simulink model "DT_V1_Transformer_Electrical_Healthy"  (R2026a)
settings: Solver=VariableStepAuto  StopTime=0.2
libraries: eeRmsMeasurement x12, nesl_utility x7, ee_lib x6, fl_lib x3

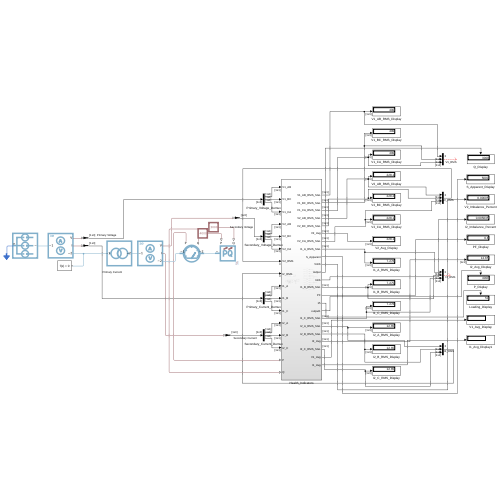
[thumbnail: Simulink's stored preview of the top-level diagram]
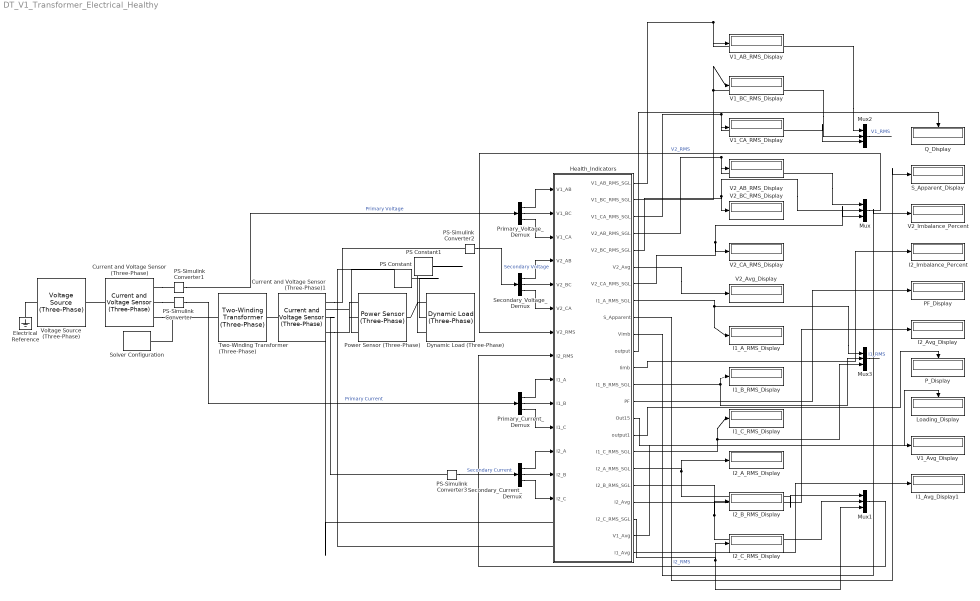
== system DT_V1_Transformer_Electrical_Healthy ==
  Current and Voltage Sensor (Three-Phase) : ee_lib/Sensors & Transducers/Current and Voltage Sensor (Three-Phase)  port_option=ee.enum.threePhasePort.composite  vMeasurementType=ee.enum.vmeasurement.ll  outputUnit=ee.enum.unit.si  SRated=100e6 A*V  VRated=24e3 V  I_specify=off  I_priority=None  I=[0, 0, 0] A  I_nominal_specify=off  I_nominal_value=1  I_nominal_unit=A  V_specify=off  V_priority=None  V=[0, 0, 0] V  V_nominal_specify=off  V_nominal_value=1  V_nominal_unit=V
  Current and Voltage Sensor (Three-Phase)1 : ee_lib/Sensors & Transducers/Current and Voltage Sensor (Three-Phase)  port_option=ee.enum.threePhasePort.composite  vMeasurementType=ee.enum.vmeasurement.ll  outputUnit=ee.enum.unit.si  SRated=100e6 A*V  VRated=24e3 V  I_specify=off  I_priority=None  I=[0, 0, 0] A  I_nominal_specify=off  I_nominal_value=1  I_nominal_unit=A  V_specify=off  V_priority=None  V=[0, 0, 0] V  V_nominal_specify=off  V_nominal_value=1  V_nominal_unit=V
  Dynamic Load (Three-Phase) : ee_lib/Passive/Dynamic Load (Three-Phase)  port_option=ee.enum.threePhasePort.composite  FRated=50 Hz  Vline_rms_min=100 V  tau=0.01 s  Vline_rms_ini=230 V  Vang_ini=0 deg  gmin=0 S
  Electrical Reference : fl_lib/Electrical/Electrical Elements/Electrical Reference
  Health_Indicators : Subsystem
  I1_A_RMS_Display : Display
  I1_Avg_Display1 : Display
  I1_B_RMS_Display : Display
  I1_C_RMS_Display : Display
  I2_A_RMS_Display : Display
  I2_Avg_Display : Display
  I2_B_RMS_Display : Display
  I2_C_RMS_Display : Display
  I2_Imbalance_Percent : Display
  Loading_Display : Display
  Mux{,1..3} (4 alike) : Mux  Inputs=3
  PF_Display : Display
  PS Constant : fl_lib/Physical Signals/Sources/PS Constant  constant=4000 W
  PS Constant1 : fl_lib/Physical Signals/Sources/PS Constant  constant=3000 A*V
  PS-Simulink Converter : nesl_utility/PS-Simulink Converter  PhysicalDomain=network_engine_domain  SubClassName=ps_output  LeftPortType=input  RightPortType=output  PseudoPeriodic=off  Frequencies=[]  VectorFormat=inherit  Unit=A  AffineConversion=off
  PS-Simulink Converter1 : nesl_utility/PS-Simulink Converter  PhysicalDomain=network_engine_domain  SubClassName=ps_output  LeftPortType=input  RightPortType=output  PseudoPeriodic=off  Frequencies=[]  VectorFormat=inherit  Unit=V  AffineConversion=off
  PS-Simulink Converter2 : nesl_utility/PS-Simulink Converter  PhysicalDomain=network_engine_domain  SubClassName=ps_output  LeftPortType=input  RightPortType=output  PseudoPeriodic=off  Frequencies=[]  VectorFormat=inherit  Unit=V  AffineConversion=off
  PS-Simulink Converter3 : nesl_utility/PS-Simulink Converter  PhysicalDomain=network_engine_domain  SubClassName=ps_output  LeftPortType=input  RightPortType=output  PseudoPeriodic=off  Frequencies=[]  VectorFormat=inherit  Unit=A  AffineConversion=off
  P_Display : Display
  Power Sensor (Three-Phase) : ee_lib/Sensors & Transducers/Power Sensor (Three-Phase)  port_option=ee.enum.threePhasePort.composite  load_type=ee.enum.passive.type_balanced.balanced  f0=60 Hz
  Primary_Current_Demux : Demux  Outputs=3
  Primary_Voltage_Demux : Demux  Outputs=3
  Q_Display : Display
  S_Apparent_Display : Display
  Secondary_Current_Demux : Demux  Outputs=3
  Secondary_Voltage_Demux : Demux  Outputs=3
  Solver Configuration : nesl_utility/Solver Configuration  PhysicalDomain=network_engine_domain  SubClassName=solver  LeftPortType=input  RightPortType=generic  Tones=[]  Harmonics=[]  SimulateNoise=off  Profile=off  UseLocalSampling=off  EnableSwitchedLinearOptims=on  FrequencyDomain=off  UseCCode=off  RelTol=0.001  AbsTol=0.001  MinStep=1e-09  ToWorkspace=off  RevertToSquareIcSolve=off  NumHomotopyIterations=100  PhasorMode=off  PhasorModeNumHarmonics=1  ConsistencySolver=NEWTON_XTOL_AFTER_FTOL  CanonicalOrdering=CANONICAL  OptimizeIntermediates=OPTIMIZED  IndexReductionMethod=DerivativeReplacement  DoDC=off  ResidualTolerance=1e-09  ConsistencyTolSource=GLOBAL  ConsistencyAbsTol=0.001  ConsistencyRelTol=0.001  ConsistencyTolFactor=0.001  UseLocalSolver=off  LocalSolverChoice=NE_BACKWARD_EULER_ADVANCER  ResolveIndetEquations=on  FunctionEvalNumThread=1  LocalSolverSampleTime=0.001  DoFixedCost=off  MaxNonlinIter=3  MaxModeIter=2  ComputeImpulses=off  ImpulseIterations=2  LinearAlgebra=auto  LinearAlgebraNumThread=0  EquationFormulation=NE_TIME_EF  DelaysMemoryBudget=1024  AutomaticFiltering=on  FilteringTimeConstant=0.001  PartitionStorageMethod=AS_NEEDED  PartitionMemoryBudget=1024  PartitionMethod=ROBUST  MultibodyUseLocalSolver=off  MultibodyLocalSolverChoice=ODE1  MultibodyLocalSolverSampleTime=0.001
  Two-Winding Transformer (Three-Phase) : ee_lib/Passive/Transformers/Two-Winding Transformer (Three-Phase)  SRated=10000 A*V  FRated=50 Hz  Winding1Connection=ee.enum.windingconnection.Yg  VRated1=400 V  Winding2Connection=ee.enum.windingconnection.Yg  VRated2=230 V  CoreType=ee.enum.coretype.threelimb  pu_Rw1=0.01  pu_Rw2=0.01  leakage_reactance_option=ee.enum.transformer_leakage.exclude  pu_Xl1=0.05  pu_Xl2=0.05  magnetizing_resistance_option=ee.enum.transformer_magnetizingResistance.exclude  pu_Rm=500  magnetizing_reactance_option=ee.enum.transformer_magnetizingReactance.exclude  saturation_option=ee.enum.transformer_saturation.exclude  pu_Xm=500  current_data=[0, .002, 1, 2]  magnetic_flux_data=[0, 1.2, 1.5, 1.51]  pu_X0=0.5  i1_specify=off  i1_priority=None  i1=[0, 0, 0] A  i1_nominal_specify=off  i1_nominal_value=1  i1_nominal_unit=A  i2_specify=off  i2_priority=None  i2=[0, 0, 0] A  i2_nominal_specify=off  i2_nominal_value=1  i2_nominal_unit=A  phi_specify=off  phi_priority=None  phi=[0, 0, 0]  phi_nominal_specify=off  phi_nominal_value=1  phi_nominal_unit=1
  V1_AB_RMS_Display : Display
  V1_Avg_Display : Display
  V1_BC_RMS_Display : Display
  V1_CA_RMS_Display : Display
  V2_AB_RMS_Display : Display
  V2_Avg_Display : Display
  V2_BC_RMS_Display : Display
  V2_CA_RMS_Display : Display
  V2_Imbalance_Percent : Display
  Voltage Source (Three-Phase) : ee_lib/Sources/Voltage Source (Three-Phase)  vline_rms=400 V  shift=0 deg  freq=50 Hz  impedance_option=0  SShortCircuit=1e6 A*V  XR=15  R=0.01 Ohm  L=3.97e-4 H  harmonic_option=0  harmonic_orders=[5, 7, 11, 13]  harmonic_ratios=[.1, .1, .1, .1]  G_parasitic=0 1/Ohm  I_specify=off  I_priority=None  I=[0, 0, 0] A  I_nominal_specify=off  I_nominal_value=1  I_nominal_unit=A
  wires:
  PS-Simulink Converter1/1 -> Primary_Voltage_Demux/1  "Primary Voltage"
  PS-Simulink Converter2/1 -> Secondary_Voltage_Demux/1  "Secondary Voltage"
  PS-Simulink Converter/1 -> Primary_Current_Demux/1  "Primary Current"
  PS-Simulink Converter3/1 -> Secondary_Current_Demux/1  "Secondary Current"
  Mux3/1 -> ?  "I1_RMS"
  Mux2/1 -> ?  "V1_RMS"
  Health_Indicators/21(I2_C_RMS_SGL) -> Mux1/3, I2_C_RMS_Display/1
  Health_Indicators/13(I1_B_RMS_SGL) -> Mux3/2, I1_B_RMS_Display/1
  Health_Indicators/17(I1_C_RMS_SGL) -> I1_C_RMS_Display/1, Mux3/3
  Health_Indicators/5(V2_BC_RMS_SGL) -> Mux/2, V2_BC_RMS_Display/1
  Health_Indicators/1(V1_AB_RMS_SGL) -> Mux2/1, V1_AB_RMS_Display/1
  Health_Indicators/18(I2_A_RMS_SGL) -> Mux1/1, I2_A_RMS_Display/1
  Health_Indicators/4(V2_AB_RMS_SGL) -> V2_AB_RMS_Display/1, Mux/1
  Health_Indicators/2(V1_BC_RMS_SGL) -> V1_BC_RMS_Display/1, Mux2/2
  Health_Indicators/19(I2_B_RMS_SGL) -> Mux1/2, I2_B_RMS_Display/1
  Health_Indicators/8(I1_A_RMS_SGL) -> I1_A_RMS_Display/1, Mux3/1
  Health_Indicators/7(V2_CA_RMS_SGL) -> Mux/3, V2_CA_RMS_Display/1
  Health_Indicators/3(V1_CA_RMS_SGL) -> V1_CA_RMS_Display/1, Mux2/3
  Primary_Voltage_Demux/1 -> Health_Indicators/1(V1_AB)
  Primary_Voltage_Demux/2 -> Health_Indicators/2(V1_BC)
  Primary_Voltage_Demux/3 -> Health_Indicators/3(V1_CA)
  Secondary_Voltage_Demux/1 -> Health_Indicators/4(V2_AB)
  Secondary_Voltage_Demux/2 -> Health_Indicators/5(V2_BC)
  Secondary_Voltage_Demux/3 -> Health_Indicators/6(V2_CA)
  Mux/1 -> Health_Indicators/7(V2_RMS)  "V2_RMS"
  Mux1/1 -> Health_Indicators/8(I2_RMS)  "I2_RMS"
  Primary_Current_Demux/1 -> Health_Indicators/9(I1_A)
  Primary_Current_Demux/2 -> Health_Indicators/10(I1_B)
  Primary_Current_Demux/3 -> Health_Indicators/11(I1_C)
  Secondary_Current_Demux/1 -> Health_Indicators/12(I2_A)
  Secondary_Current_Demux/2 -> Health_Indicators/13(I2_B)
  Secondary_Current_Demux/3 -> Health_Indicators/14(I2_C)
  Health_Indicators/6(V2_Avg) -> V2_Avg_Display/1
  Health_Indicators/9(S_Apparent) -> S_Apparent_Display/1
  Health_Indicators/10(Vimb) -> V2_Imbalance_Percent/1
  Health_Indicators/11(output) -> Q_Display/1
  Health_Indicators/12(Iimb) -> I2_Imbalance_Percent/1
  Health_Indicators/14(PF) -> PF_Display/1
  Health_Indicators/15(Out15) -> Loading_Display/1
  Health_Indicators/16(output1) -> P_Display/1
  Health_Indicators/20(I2_Avg) -> I2_Avg_Display/1
  Health_Indicators/22(V1_Avg) -> V1_Avg_Display/1
  Health_Indicators/23(I1_Avg) -> I1_Avg_Display1/1
  connections:
  Voltage Source (Three-Phase)/LConn1 -- Electrical Reference/LConn1
  PS Constant/RConn1 -- Dynamic Load (Three-Phase)/LConn2
  PS Constant1/RConn1 -- Dynamic Load (Three-Phase)/LConn3
  Current and Voltage Sensor (Three-Phase)/LConn1 -- Voltage Source (Three-Phase)/RConn1
  Current and Voltage Sensor (Three-Phase)/RConn3 -- Solver Configuration/RConn1 -- Two-Winding Transformer (Three-Phase)/LConn1
  Current and Voltage Sensor (Three-Phase)/RConn1 -- PS-Simulink Converter1/LConn1
  Current and Voltage Sensor (Three-Phase)/RConn2 -- PS-Simulink Converter/LConn1
  Current and Voltage Sensor (Three-Phase)1/RConn1 -- PS-Simulink Converter2/LConn1
  Current and Voltage Sensor (Three-Phase)1/RConn2 -- PS-Simulink Converter3/LConn1
  Current and Voltage Sensor (Three-Phase)1/LConn1 -- Two-Winding Transformer (Three-Phase)/RConn1
  Power Sensor (Three-Phase)/LConn2 -- Health_Indicators/LConn1
  Health_Indicators/LConn2 -- Power Sensor (Three-Phase)/LConn3
  Dynamic Load (Three-Phase)/LConn1 -- Power Sensor (Three-Phase)/RConn1
  Current and Voltage Sensor (Three-Phase)1/RConn3 -- Power Sensor (Three-Phase)/LConn1

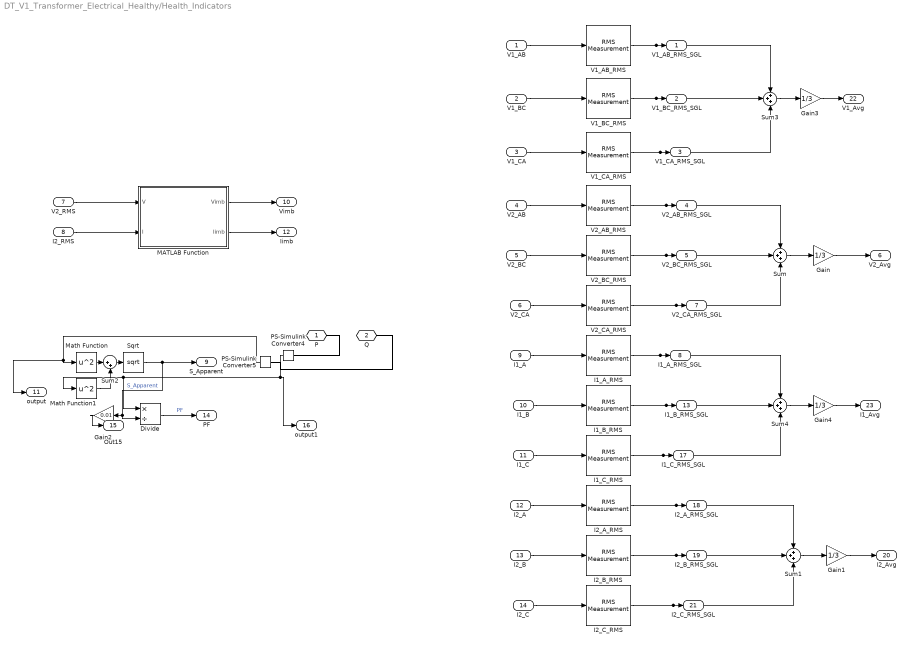
== system DT_V1_Transformer_Electrical_Healthy/Health_Indicators ==
  V1_AB : Inport
  V1_BC : Inport  Port=2
  V1_CA : Inport  Port=3
  V2_AB : Inport  Port=4
  V2_BC : Inport  Port=5
  V2_CA : Inport  Port=6
  V2_RMS : Inport  Port=7
  I2_RMS : Inport  Port=8
  I1_A : Inport  Port=9
  I1_B : Inport  Port=10
  I1_C : Inport  Port=11
  I2_A : Inport  Port=12
  I2_B : Inport  Port=13
  I2_C : Inport  Port=14
  Divide : Product  Inputs=*/
  Gain{,1,3..4} (4 alike) : Gain  Gain=1/3
  Gain2 : Gain  Gain=0.01
  I1_A_RMS : eeRmsMeasurement/RMS Measurement  LabelModeActiveChoice=Total  F=50  SpecifyHarmonics=off  K=[0 1 2]  Ts=0
      settings: LibrarySourceBlock=|
      | ee_sl_lib/Measurements/RMS
      | Measurement
  I1_B_RMS : eeRmsMeasurement/RMS Measurement  LabelModeActiveChoice=Total  F=50  SpecifyHarmonics=off  K=[0 1 2]  Ts=0
      settings: LibrarySourceBlock=|
      | ee_sl_lib/Measurements/RMS
      | Measurement
  I1_C_RMS : eeRmsMeasurement/RMS Measurement  LabelModeActiveChoice=Total  F=50  SpecifyHarmonics=off  K=[0 1 2]  Ts=0
      settings: LibrarySourceBlock=|
      | ee_sl_lib/Measurements/RMS
      | Measurement
  I2_A_RMS : eeRmsMeasurement/RMS Measurement  LabelModeActiveChoice=Total  F=50  SpecifyHarmonics=off  K=[0 1 2]  Ts=0
      settings: LibrarySourceBlock=|
      | ee_sl_lib/Measurements/RMS
      | Measurement
  I2_B_RMS : eeRmsMeasurement/RMS Measurement  LabelModeActiveChoice=Total  F=50  SpecifyHarmonics=off  K=[0 1 2]  Ts=0
      settings: LibrarySourceBlock=|
      | ee_sl_lib/Measurements/RMS
      | Measurement
  I2_C_RMS : eeRmsMeasurement/RMS Measurement  LabelModeActiveChoice=Total  F=50  SpecifyHarmonics=off  K=[0 1 2]  Ts=0
      settings: LibrarySourceBlock=|
      | ee_sl_lib/Measurements/RMS
      | Measurement
  MATLAB Function : MATLAB Function  TreatAsAtomicUnit=on
  Math Function : Math  Operator=square
  Math Function1 : Math  Operator=square
  PS-Simulink Converter4 : nesl_utility/PS-Simulink Converter  PhysicalDomain=network_engine_domain  SubClassName=ps_output  LeftPortType=input  RightPortType=output  PseudoPeriodic=off  Frequencies=[]  VectorFormat=inherit  Unit=W  AffineConversion=off
  PS-Simulink Converter5 : nesl_utility/PS-Simulink Converter  PhysicalDomain=network_engine_domain  SubClassName=ps_output  LeftPortType=input  RightPortType=output  PseudoPeriodic=off  Frequencies=[]  VectorFormat=inherit  Unit=W  AffineConversion=off
  Sqrt : Sqrt
  Sum{,1,3..4} (4 alike) : Sum  Inputs=+++
  Sum2 : Sum  Inputs=|++
  V1_AB_RMS : eeRmsMeasurement/RMS Measurement  LabelModeActiveChoice=Total  F=50  SpecifyHarmonics=off  K=[0 1 2]  Ts=0
      settings: LibrarySourceBlock=|
      | ee_sl_lib/Measurements/RMS
      | Measurement
  V1_BC_RMS : eeRmsMeasurement/RMS Measurement  LabelModeActiveChoice=Total  F=50  SpecifyHarmonics=off  K=[0 1 2]  Ts=0
      settings: LibrarySourceBlock=|
      | ee_sl_lib/Measurements/RMS
      | Measurement
  V1_CA_RMS : eeRmsMeasurement/RMS Measurement  LabelModeActiveChoice=Total  F=50  SpecifyHarmonics=off  K=[0 1 2]  Ts=0
      settings: LibrarySourceBlock=|
      | ee_sl_lib/Measurements/RMS
      | Measurement
  V2_AB_RMS : eeRmsMeasurement/RMS Measurement  LabelModeActiveChoice=Total  F=50  SpecifyHarmonics=off  K=[0 1 2]  Ts=0
      settings: LibrarySourceBlock=|
      | ee_sl_lib/Measurements/RMS
      | Measurement
  V2_BC_RMS : eeRmsMeasurement/RMS Measurement  LabelModeActiveChoice=Total  F=50  SpecifyHarmonics=off  K=[0 1 2]  Ts=0
      settings: LibrarySourceBlock=|
      | ee_sl_lib/Measurements/RMS
      | Measurement
  V2_CA_RMS : eeRmsMeasurement/RMS Measurement  LabelModeActiveChoice=Total  F=50  SpecifyHarmonics=off  K=[0 1 2]  Ts=0
      settings: LibrarySourceBlock=|
      | ee_sl_lib/Measurements/RMS
      | Measurement
  P : PMIOPort  Side=Left
  Q : PMIOPort  Port=2  Side=Left
  V1_AB_RMS_SGL : Outport
  V1_BC_RMS_SGL : Outport  Port=2
  V1_CA_RMS_SGL : Outport  Port=3
  V2_AB_RMS_SGL : Outport  Port=4
  V2_BC_RMS_SGL : Outport  Port=5
  V2_Avg : Outport  Port=6
  V2_CA_RMS_SGL : Outport  Port=7
  I1_A_RMS_SGL : Outport  Port=8
  S_Apparent : Outport  Port=9
  Vimb : Outport  Port=10
  output : Outport  Port=11
  Iimb : Outport  Port=12
  I1_B_RMS_SGL : Outport  Port=13
  PF : Outport  Port=14
  Out15 : Outport  Port=15
  output1 : Outport  Port=16
  I1_C_RMS_SGL : Outport  Port=17
  I2_A_RMS_SGL : Outport  Port=18
  I2_B_RMS_SGL : Outport  Port=19
  I2_Avg : Outport  Port=20
  I2_C_RMS_SGL : Outport  Port=21
  V1_Avg : Outport  Port=22
  I1_Avg : Outport  Port=23
  wires:
  V1_AB/1 -> V1_AB_RMS/1
  V2_RMS/1 -> MATLAB Function/1(V)
  V1_CA_RMS/1 -> Sum3/3, V1_CA_RMS_SGL/1
  I2_A_RMS/1 -> Sum1/1, I2_A_RMS_SGL/1
  V2_BC/1 -> V2_BC_RMS/1
  I1_B_RMS/1 -> Sum4/2, I1_B_RMS_SGL/1
  MATLAB Function/2(Iimb) -> Iimb/1
  I2_B_RMS/1 -> Sum1/2, I2_B_RMS_SGL/1
  I1_B/1 -> I1_B_RMS/1
  I2_A/1 -> I2_A_RMS/1
  I2_C/1 -> I2_C_RMS/1
  V1_BC_RMS/1 -> Sum3/2, V1_BC_RMS_SGL/1
  Sqrt/1 -> S_Apparent/1, Divide/2, Gain2/1  "S_Apparent"
  I1_C/1 -> I1_C_RMS/1
  Divide/1 -> PF/1  "PF"
  PS-Simulink Converter4/1 -> output1/1, Divide/1, Math Function1/1
  V2_CA_RMS/1 -> Sum/3, V2_CA_RMS_SGL/1
  Gain/1 -> V2_Avg/1
  V1_CA/1 -> V1_CA_RMS/1
  V1_BC/1 -> V1_BC_RMS/1
  V2_AB/1 -> V2_AB_RMS/1
  I1_C_RMS/1 -> Sum4/3, I1_C_RMS_SGL/1
  Sum/1 -> Gain/1
  V1_AB_RMS/1 -> V1_AB_RMS_SGL/1, Sum3/1
  I2_B/1 -> I2_B_RMS/1
  I1_A_RMS/1 -> Sum4/1, I1_A_RMS_SGL/1
  MATLAB Function/1(Vimb) -> Vimb/1
  Gain1/1 -> I2_Avg/1
  I2_C_RMS/1 -> Sum1/3, I2_C_RMS_SGL/1
  I2_RMS/1 -> MATLAB Function/2(I)
  Math Function1/1 -> Sum2/2
  Gain2/1 -> Out15/1
  V2_AB_RMS/1 -> Sum/1, V2_AB_RMS_SGL/1
  I1_A/1 -> I1_A_RMS/1
  V2_CA/1 -> V2_CA_RMS/1
  V2_BC_RMS/1 -> Sum/2, V2_BC_RMS_SGL/1
  Math Function/1 -> Sum2/1
  PS-Simulink Converter5/1 -> output/1, Math Function/1
  Sum1/1 -> Gain1/1
  Sum2/1 -> Sqrt/1
  Sum3/1 -> Gain3/1
  Gain3/1 -> V1_Avg/1
  Sum4/1 -> Gain4/1
  Gain4/1 -> I1_Avg/1
  connections:
  P/RConn1 -- PS-Simulink Converter4/LConn1
  PS-Simulink Converter5/LConn1 -- Q/RConn1

== matlab function DT_V1_Transformer_Electrical_Healthy/Health_Indicators/MATLAB Function ==
  data: V input double size=[1 3]; Vimb output double size=[1 1]; I input double size=[1 3]; Iimb output double size=[1 1]
function [Vimb, Iimb] = phase_imbalance(V, I)

Vavg = sum(V) / 3;
Iavg = sum(I) / 3;

Vdev = abs(V - Vavg);
Idev = abs(I - Iavg);

Vimb = max(Vdev) / Vavg * 100;
Iimb = max(Idev) / Iavg * 100;
